simulink model "SimulationMain"  (R2023b)
settings: Solver=FixedStepAuto  StartTime=0.0  StopTime=Inf  RelTol=1e-3
undefined symbols (not defined in the file): ADC_VMax, ADC_VMin, CurrentSensor_Bias, CurrentSensor_Gain, DC_V, DiscIntNeverNeededParam, DoorStairOutTime1, DoorStairOutTime2, FloorHeight, FloorStairOut, FloorTimeStairOut, IO397, Omega2RPM, Pulley, StairOutTime1, StairOutTime2
libraries: fl_lib x10, ee_lib x10, nesl_utility x8, mcbplantlib x1, speedgoatlib_fpga x1, speedgoatlib_fpga_analog_io x1, speedgoatlib_fpga_quadrature x1, speedgoatlib_fpga_pwm x1
settings Model: DataDictionary=Data_GeneralDefinition.sldd  Creator=rodri  LastModifiedBy=rodri
settings SolverCC: ConcurrentTasks=on  PositivePriorityOrder=on
settings OptimizationCC: BlockReduction=off  OptimizeBlockIOStorage=off
settings DebuggingCC: TasksWithSamePriorityMsg=none
settings HardwareCC: ProdBitPerLong=64  ProdLongLongMode=on  ProdHWDeviceType=Intel->x86-64 (Linux 64)
settings ModelReferenceCC: ModelReferenceNumInstancesAllowed=Single
settings RTWCC: Description=Simulink Real-Time  SystemTargetFile=slrealtime.tlc  TemplateMakefile=slrealtime_default_tmf  Toolchain=Simulink Real-Time Toolchain  BuildConfiguration=Faster Runs  CodeExecutionProfiling=on  TargetLang=C++
settings ExplorerConfigSet: SimMechanicsOpenEditorOnUpdate=off

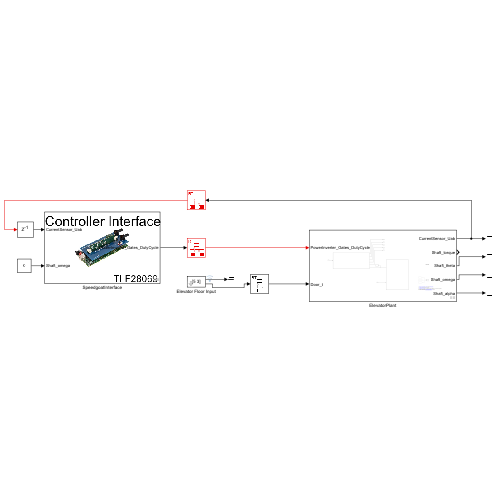
[thumbnail: Simulink's stored preview of the top-level diagram]
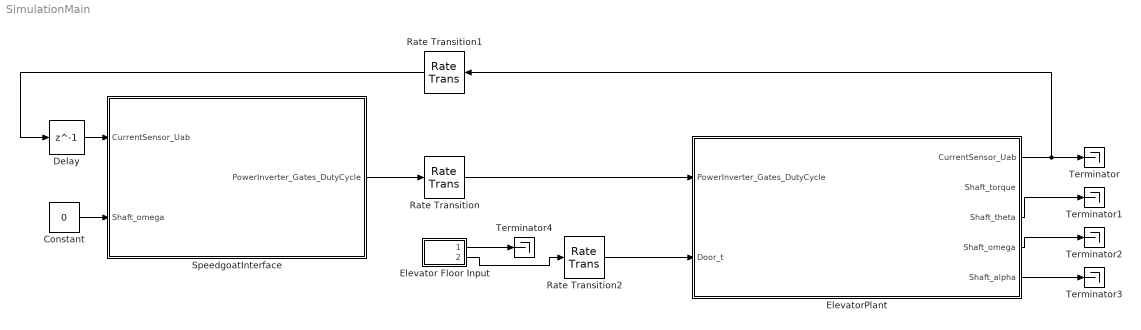
== system SimulationMain ==
  Constant : Constant  Value=0  SampleTime=-1
  Delay : Delay  DelayLength=1
  Elevator Floor Input : Subsystem  mask(Elevator Floors Input){FloorNums=[5 3]}
      mask prompts: FloorNums "Enter Floor Numbers"
      mask help:
      | Provide the floor numbers (1 to 7) for the elevator. This should be a (1 x n) vector. (n<=3)
      |
      | For example, an input of [4 2] means the elevator will go to the 4th Floor first and then the 2nd Floor.
      mask init:
      | if ~isrow(str2num(get_param(gcb,'FloorNums')))
      |     error('Input should be a row vector');
      | end
      | 
      | if length(str2num(get_param(gcb,'FloorNums')))>3
      |     error('Length of input row vector should not be greater then 3');
      | end
      | 
      | if any(str2num(get_param(gcb,'FloorNums'))>7)
      |     error('Elevator can not go above 7 floors for this system');
      | end
      | 
      | if any(str2num(get_param(gcb,'FloorNums'))<=0)
      |     error('Elevator floor input should be greater then 0');
      | end
      mask Display: disp(get_param(gcb,'FloorNums'));
  ElevatorPlant : Subsystem
  Rate Transition : RateTransition
  Rate Transition1 : RateTransition
  Rate Transition2 : RateTransition
  SpeedgoatInterface : Subsystem
  Terminator{,1..4} (5 alike) : Terminator
  wires:
  SpeedgoatInterface/1(PowerInverter_Gates_DutyCycle) -> Rate Transition/1
  Constant/1 -> SpeedgoatInterface/2(Shaft_omega)
  ElevatorPlant/1(CurrentSensor_Uab) -> Rate Transition1/1, Terminator/1
  ElevatorPlant/3(Shaft_theta) -> Terminator1/1
  ElevatorPlant/4(Shaft_omega) -> Terminator2/1
  ElevatorPlant/5(Shaft_alpha) -> Terminator3/1
  Delay/1 -> SpeedgoatInterface/1(CurrentSensor_Uab)
  Rate Transition/1 -> ElevatorPlant/1(PowerInverter_Gates_DutyCycle)
  Rate Transition1/1 -> Delay/1
  Elevator Floor Input/2(DoorOperationTimes) -> Rate Transition2/1
  Elevator Floor Input/1(MotorMotion) -> Terminator4/1
  Rate Transition2/1 -> ElevatorPlant/2(Door_t)

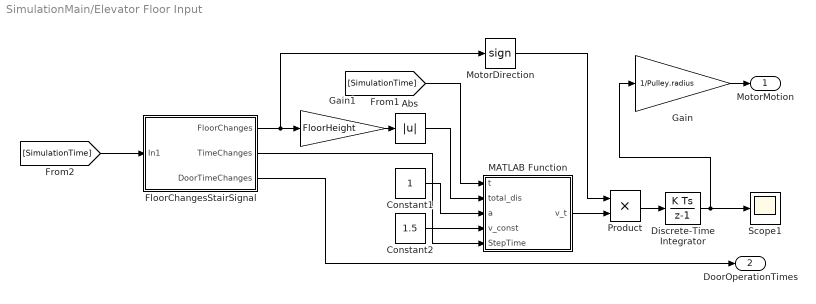
== system SimulationMain/Elevator Floor Input ==
  Abs : Abs  SaturateOnIntegerOverflow=off
  Constant1 : Constant  SampleTime=-1
  Constant2 : Constant  Value=1.5  SampleTime=-1
  Discrete-Time Integrator : DiscreteIntegrator  SampleTime=-1  ICPrevOutput=DiscIntNeverNeededParam  ICPrevScaledInput=DiscIntNeverNeededParam
  FloorChangesStairSignal : Subsystem  mask{FloorNums=FloorNums}
      mask prompts: FloorNums "Enter Floor Nums for Elevator"
      mask init:
      | [FloorStairOut,FloorTimeStairOut,StairOutTime1,StairOutTime2,DoorStairOutTime1,DoorStairOutTime2]...
      |  = getLookUpTableData(FloorNums);
  Gain : Gain  Gain=1/Pulley.radius
  Gain1 : Gain  Gain=FloorHeight
  MATLAB Function : MATLAB Function  TreatAsAtomicUnit=on
  MotorDirection : Signum
  Product : Product
  Scope1 : Scope
  MotorMotion : Outport  VectorParamsAs1DForOutWhenUnconnected=off
  DoorOperationTimes : Outport  Port=2  VectorParamsAs1DForOutWhenUnconnected=off
  wires:
  FloorChangesStairSignal/3(DoorTimeChanges) -> DoorOperationTimes/1
  Abs/1 -> MATLAB Function/2(total_dis)
  FloorChangesStairSignal/1(FloorChanges) -> MotorDirection/1, Gain1/1
  FloorChangesStairSignal/2(TimeChanges) -> MATLAB Function/5(StepTime)
  MATLAB Function/1(v_t) -> Product/2
  Product/1 -> Discrete-Time Integrator/1
  MotorDirection/1 -> Product/1
  Gain/1 -> MotorMotion/1
  Gain1/1 -> Abs/1
  [SimulationTime] -> MATLAB Function/1(t)
  Constant1/1 -> MATLAB Function/3(a)
  Constant2/1 -> MATLAB Function/4(v_const)
  Discrete-Time Integrator/1 -> Scope1/1, Gain/1
  [SimulationTime] -> FloorChangesStairSignal/1(In1)

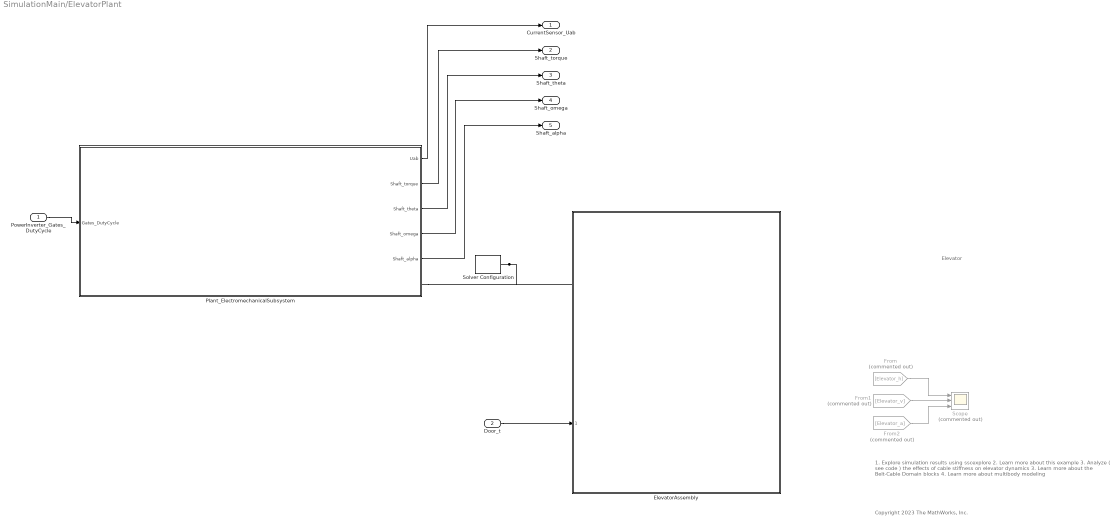
== system SimulationMain/ElevatorPlant ==
  note: 1. Explore simulation results using sscexplore
      | 2. Learn more about this example
      | 3. Analyze ( see code ) the effects of cable stiffness on elevator dynamics
      | 3. Learn more about the Belt-Cable Domain blocks
      | 4. Learn more about multibody modeling
  note: Elevator
  note: Copyright 2023 The MathWorks, Inc.
  PowerInverter_Gates_DutyCycle : Inport
  Door_t : Inport  Port=2
  ElevatorAssembly : Subsystem  ReferencedSubsystem=ElevatorAssembly
      settings: PortSchema="{\"entries\":[{\"content\":{\"sides\":[{\"content\":{\"connectorIds\":[\"LConn1\",\"In1\"]},\"type\":\"ConnectorPlacement.EquallySpacedRectSide\",\"uuid\":\"d6cdcc45-76f5-4e8f-aa72-f7931a260e9d\"},{\"content\":{\"side\":\"RIGHT\"},\"type\":\"ConnectorPlacement.EquallySpacedRectSide\",\"uuid\":\"7886d4e3-3d61-4781-ae6a-17f03b8e636c\"},{\"content\":{\"side\":\"TOP\"},\"type\":\"ConnectorPlacement.EquallySpacedRectSide\",\"uuid\":\"a03356aa-ba1a-42a9-a233-3323839a0ec6\"}]},\"type\":\"ConnectorPlacement.EquallySpacedConnector\",\"uuid\":\"80b5650e-2a4d-4b3a-8116-45d32f4901f0\"}],\"packageUris\":[\"http://schema.mathworks.com/mf0/Connector/R2020b\"],\"version\":\"1.0\"}"
  From : From  Commented=on  GotoTag=Elevator_h  TagVisibility=global
  From1 : From  Commented=on  GotoTag=Elevator_v  TagVisibility=global
  From2 : From  Commented=on  GotoTag=Elevator_a  TagVisibility=global
  Plant_ElectromechanicalSubsystem : Subsystem
  Scope : Scope  Commented=on  NumInputPorts=3
  Solver Configuration : nesl_utility/Solver Configuration  PhysicalDomain=network_engine_domain  SubClassName=solver  LeftPortType=input  RightPortType=generic  Tones=[]  Harmonics=[]  SimulateNoise=off  Profile=off  UseLocalSampling=off  EnableSwitchedLinearOptims=on  FrequencyDomain=off  UseCCode=off  RelTol=0.001  AbsTol=0.001  MinStep=1e-09  ToWorkspace=off  RevertToSquareIcSolve=off  NumHomotopyIterations=100  PhasorMode=off  PhasorModeNumHarmonics=1  ConsistencySolver=NEWTON_XTOL_AFTER_FTOL  IndexReductionMethod=DerivativeReplacement  DoDC=off  ResidualTolerance=1e-09  ConsistencyTolSource=GLOBAL  ConsistencyAbsTol=0.001  ConsistencyRelTol=0.001  ConsistencyTolFactor=0.001  UseLocalSolver=on  LocalSolverChoice=NE_BACKWARD_EULER_ADVANCER  ResolveIndetEquations=on  FunctionEvalNumThread=1  LocalSolverSampleTime=0.002  DoFixedCost=on  MaxNonlinIter=3  MaxModeIter=2  ComputeImpulses=off  ImpulseIterations=2  LinearAlgebra=auto  LinearAlgebraNumThread=0  EquationFormulation=NE_TIME_EF  DelaysMemoryBudget=1024  AutomaticFiltering=on  FilteringTimeConstant=0.001  PartitionStorageMethod=AS_NEEDED  PartitionMemoryBudget=1024  PartitionMethod=ROBUST  MultibodyUseLocalSolver=off  MultibodyLocalSolverChoice=ODE1  MultibodyLocalSolverSampleTime=0.001
  CurrentSensor_Uab : Outport
  Shaft_torque : Outport  Port=2
  Shaft_theta : Outport  Port=3
  Shaft_omega : Outport  Port=4
  Shaft_alpha : Outport  Port=5
  wires:
  Plant_ElectromechanicalSubsystem/5(Shaft_alpha) -> Shaft_alpha/1
  Plant_ElectromechanicalSubsystem/4(Shaft_omega) -> Shaft_omega/1
  Plant_ElectromechanicalSubsystem/3(Shaft_theta) -> Shaft_theta/1
  Plant_ElectromechanicalSubsystem/2(Shaft_torque) -> Shaft_torque/1
  Plant_ElectromechanicalSubsystem/1(Uab) -> CurrentSensor_Uab/1
  PowerInverter_Gates_DutyCycle/1 -> Plant_ElectromechanicalSubsystem/1(Gates_DutyCycle)
  From/1 -> Scope/1
  From1/1 -> Scope/2
  From2/1 -> Scope/3
  Door_t/1 -> ElevatorAssembly/1
  connections:
  Solver Configuration/RConn1 -- ElevatorAssembly/LConn1 -- Plant_ElectromechanicalSubsystem/RConn1

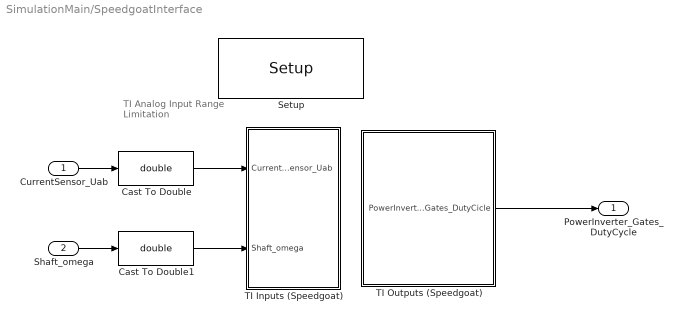
== system SimulationMain/SpeedgoatInterface ==
  note: TI Analog Input Range Limitation
  CurrentSensor_Uab : Inport  OutDataTypeStr=double  PortDimensions=2
  Shaft_omega : Inport  Port=2  OutDataTypeStr=double  PortDimensions=1
  Cast To Double : DataTypeConversion  OutMin=ADC_VMin  OutMax=ADC_VMax  OutDataTypeStr=double  SaturateOnIntegerOverflow=off  RndMeth=Floor
  Cast To Double1 : DataTypeConversion  OutDataTypeStr=double  SaturateOnIntegerOverflow=off  RndMeth=Floor
  Setup : speedgoatlib_fpga/Setup/Setup  board=IO397-50k  id=1  device_id=1  frontIO=None  rearIO=None  bitstreamFile=speedgoat_IO397_HIL.mat  rev=7.100000  timestamp_string=04/06/24 08:23:17  fpgaFreq=75 MHz  fpgaTick=13.33 ns  ProgSpiFlash=off  ProgBPIFlash=off  pciSlot=-1  useFpgaDmaController=off  PullRPort0=pull-up 3.3V  VioPort0=3.3V  PullRPort1=pull-up 3.3V  VioPort1=3.3V  PullRPort2=pull-up 3.3V  VioPort2=3.3V  PullRPort3=pull-up 3.3V  VioPort3=3.3V  PullRPort4=pull-up 3.3V  VioPort4=3.3V  PullRPort5=pull-up 3.3V  VioPort5=3.3V  PullRPort6=pull-up 3.3V  VioPort6=3.3V  diffLineTermination_rear1=on  diffLineTermination_rear2=on  diffLineTermination_rear3=on  diffLineTermination_rear4=on  diffLineTermination_rear5=on  diffLineTermination_rear6=on  diffLineTermination_rear7=on  diffLineTermination_rear8=on  PullRPort15=pull-up 3.3V  PullRPort31=pull-up 3.3V  PullRPort47=pull-up 3.3V  PullRPort63=pull-up 3.3V  diffLineTermination_1=on  diffLineTermination_2=on  diffLineTermination_3=on  diffLineTermination_4=on  diffLineTermination_5=on  diffLineTermination_6=on  diffLineTermination_7=on  diffLineTermination_8=on  diffLineTermination_9=on  diffLineTermination_10=on  diffLineTermination_11=on  diffLineTermination_12=on  diffLineTermination_13=on  diffLineTermination_14=on  diffLineTermination_15=on  diffLineTermination_16=on  diffLineTermination_17=on  diffLineTermination_18=on  diffLineTermination_19=on  diffLineTermination_20=on  diffLineTermination_21=on  diffLineTermination_22=on  diffLineTermination_23=on  diffLineTermination_24=on  diffLineTermination_25=on  diffLineTermination_26=on  diffLineTermination_27=on  diffLineTermination_28=on  diffLineTermination_29=on  diffLineTermination_30=on  diffLineTermination_31=on  diffLineTermination_32=on  Vo_36x_1=3.3V  Vi_Pull_36x_1=Floating  Vo_36x_2=3.3V  Vi_Pull_36x_2=Floating  Vo_36x_3=3.3V  Vi_Pull_36x_3=Floating  Vo_36x_4=3.3V  Vi_Pull_36x_4=Floating  Vo_36x_5=3.3V  Vi_Pull_36x_5=Floating  Vo_36x_6=3.3V  Vi_Pull_36x_6=Floating  Vo_36x_7=3.3V  Vi_Pull_36x_7=Floating  Vo_36x_8=3.3V  Vi_Pull_36x_8=Floating  Vo_36x_9_16=3.3V  Vi_Pull_36x_9_16=Floating  Vo_36x_17_24=3.3V  Vi_Pull_36x_17_24=Floating  Vo_36x_25_32=3.3V  Vi_Pull_36x_25_32=Floating  Vo_36x_33_40=3.3V  Vi_Pull_36x_33_40=Floating  Vo_36x_41_48=3.3V  Vi_Pull_36x_41_48=Floating  Vo_36x_49_56=3.3V  Vi_Pull_36x_49_56=Floating  Vo_36x_57_64=3.3V  Vi_Pull_36x_57_64=Floating
      settings: SourceProductName=Simulink Real-Time: Speedgoat I/O Blockset
  TI Inputs (Speedgoat) : Subsystem
  TI Outputs (Speedgoat) : Subsystem
  PowerInverter_Gates_DutyCycle : Outport  OutDataTypeStr=double  PortDimensions=6
  wires:
  Cast To Double1/1 -> TI Inputs (Speedgoat)/2(Shaft_omega)
  CurrentSensor_Uab/1 -> Cast To Double/1
  Shaft_omega/1 -> Cast To Double1/1
  Cast To Double/1 -> TI Inputs (Speedgoat)/1(CurrentSensor_Uab)
  TI Outputs (Speedgoat)/1(PowerInverter_Gates_DutyCicle) -> PowerInverter_Gates_DutyCycle/1

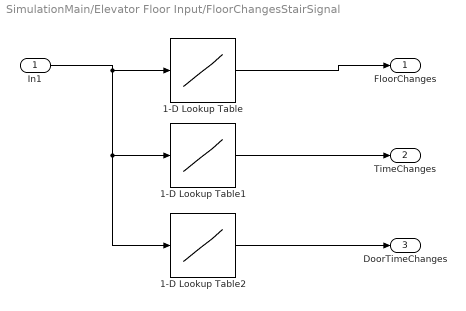
== system SimulationMain/Elevator Floor Input/FloorChangesStairSignal ==
  In1 : Inport
  1-D Lookup Table : Lookup_n-D  NumberOfTableDimensions=1  BreakpointsForDimension1=FloorTimeStairOut  BreakpointsForDimension1FirstPoint=2  Table=FloorStairOut  ExtrapMethod=Clip  UseLastTableValue=on  InternalRulePriority=Speed  RndMeth=Nearest
  1-D Lookup Table1 : Lookup_n-D  NumberOfTableDimensions=1  BreakpointsForDimension1=StairOutTime2  BreakpointsForDimension1FirstPoint=2  Table=StairOutTime1  ExtrapMethod=Clip  UseLastTableValue=on  InternalRulePriority=Speed  RndMeth=Nearest
  1-D Lookup Table2 : Lookup_n-D  NumberOfTableDimensions=1  BreakpointsForDimension1=DoorStairOutTime2  BreakpointsForDimension1FirstPoint=2  Table=DoorStairOutTime1  ExtrapMethod=Clip  UseLastTableValue=on  InternalRulePriority=Speed  RndMeth=Nearest
  FloorChanges : Outport  VectorParamsAs1DForOutWhenUnconnected=off
  TimeChanges : Outport  Port=2  VectorParamsAs1DForOutWhenUnconnected=off
  DoorTimeChanges : Outport  Port=3  VectorParamsAs1DForOutWhenUnconnected=off
  wires:
  In1/1 -> 1-D Lookup Table2/1, 1-D Lookup Table1/1, 1-D Lookup Table/1
  1-D Lookup Table/1 -> FloorChanges/1
  1-D Lookup Table1/1 -> TimeChanges/1
  1-D Lookup Table2/1 -> DoorTimeChanges/1

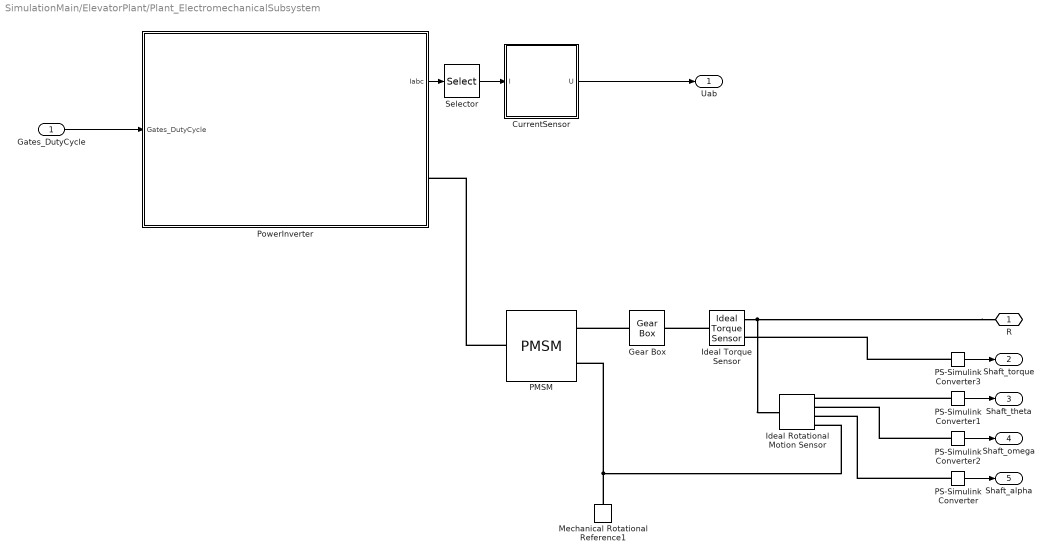
== system SimulationMain/ElevatorPlant/Plant_ElectromechanicalSubsystem ==
  Gates_DutyCycle : Inport
  CurrentSensor : Subsystem
  Gear Box : fl_lib/Mechanical/Mechanisms/Gear Box  ratio=10  t_in_specify=off  t_in_priority=None  t_in=0 N*m  t_in_nominal_specify=off  t_in_nominal_unit=N*m  t_in_nominal_value=1  t_out_specify=off  t_out_priority=None  t_out=0 N*m  t_out_nominal_specify=off  t_out_nominal_unit=N*m  t_out_nominal_value=1
  Ideal Rotational Motion Sensor : fl_lib/Mechanical/Mechanical Sensors/Ideal Rotational Motion Sensor  reference=foundation.enum.MeasurementReference.difference  acceleration_port=true  velocity_port=true  position_port=true  wrap_angle=false  offset=0 rad
      settings: InternalSimscapePortConfiguration="{\"Bottom\":[],\"Left\":[{\"id\":\"R\",\"label\":\"R\",\"type\":\"foundation.mechanical.rotational.rotational\"}],\"Right\":[{\"id\":\"C\",\"label\":\"C\",\"type\":\"foundation.mechanical.rotational.rotational\"},{\"id\":\"alpha\",\"label\":\"α\",\"type\":\"output\"},{\"id\":\"W\",\"label\":\"W\",\"type\":\"output\"},{\"id\":\"A\",\"label\":\"A\",\"type\":\"output\"}],\"Top\":[]}"
  Ideal Torque Sensor : fl_lib/Mechanical/Mechanical Sensors/Ideal Torque Sensor
  Mechanical Rotational Reference1 : fl_lib/Mechanical/Rotational Elements/Mechanical Rotational Reference
  PMSM : ee_lib/Electromechanical/Permanent Magnet/PMSM  Tag={'toolbox/physmod/elec/library/m/ee_lib_parts';'Electromechanical/Permanent_Magnet/PMSM/Siemens/x1FT7108_5AC7.xml'}  port_option=ee.enum.threePhasePort.composite  winding_type=ee.enum.statorconnection.wye  machine_param=ee.enum.pmsm.parameterization.constant  nPolePairs=5  pmflux_param=ee.enum.pmflux.fluxlinkage  pm_flux_linkage=0.270554790028086 Wb  torque_constant=1.35277395014043 N*m/A  back_emf_constant=1.35277395014043 V/(rad/s)  stator_param=ee.enum.statorparam.LdLqL0  Ld=0.0031 H  Lq=0.0031 H  idVec=[-200 0 200] % Parameter not set A  iqVec=[-200 0 200] % Parameter not set A  LdMatrix=[0.0002 0.0002 0.0002;0.0002 0.0002 0.0002;0.0002 0.0002 0.0002] % Parameter not set H  LqMatrix=[0.0002 0.0002 0.0002;0.0002 0.0002 0.0002;0.0002 0.0002 0.0002] % Parameter not set H  PmMatrix=[0.1 0.1 0.1;0.1 0.1 0.1;0.1 0.1 0.1] Wb  ktMatrix=[0.18 0.18 0.18;0.18 0.18 0.18;0.18 0.18 0.18] N*m/A  keMatrix=[0.18 0.18 0.18;0.18 0.18 0.18;0.18 0.18 0.18] % Parameter not set V/(rad/s)  L0=[] % Parameter not set H  Ls=0.0002 H  Lm=-2e-05 H  Ms=2e-05 H  Rs=0.111 Ohm  zero_sequence=ee.enum.park.zerosequence.exclude  axes_param=ee.enum.rotorangle.daxis  loss_param=ee.enum.ironloss.none  losses_oc=[0 0 0] % Parameter not set W  losses_sc=[0 0 0] % Parameter not set W  f_losses=60 % Parameter not set Hz  Isc_losses=95 % Parameter not set A  J=0.0248 kg*m^2  lam=0 % Parameter not set N*m/(rad/s)  i_d_specify=off  i_d_priority=None  i_d=0 A  i_d_nominal_specify=off  i_d_nominal_unit=A  i_d_nominal_value=1  i_q_specify=off  i_q_priority=None  i_q=0 A  i_q_nominal_specify=off  i_q_nominal_unit=A  i_q_nominal_value=1  torque_specify=off  torque_priority=None  torque=0 N*m  torque_nominal_specify=off  torque_nominal_unit=N*m  torque_nominal_value=1  angular_velocity_specify=off  angular_velocity_priority=High  angular_velocity=0 rpm  angular_velocity_nominal_specify=off  angular_velocity_nominal_unit=rpm  angular_velocity_nominal_value=1  angular_position_specify=off  angular_position_priority=High  angular_position=0 deg  angular_position_nominal_specify=off  angular_position_nominal_unit=deg  angular_position_nominal_value=1  alpha=3.93e-3 1/K  alpha_flux=-0.001 1/K  Tmeas=298.15 K  stator_thermal_mass=100 J/K  rotor_thermal_mass=200 J/K  Rm_percent_rotor=90  Rd_percent_rotor=30  temperatureA_specify=off  temperatureA_priority=High  temperatureA=25 degC  temperatureA_nominal_specify=off  temperatureA_nominal_unit=degC  temperatureA_nominal_value=1  temperatureB_specify=off  temperatureB_priority=High  temperatureB=25 degC  temperatureB_nominal_specify=off  temperatureB_nominal_unit=degC  temperatureB_nominal_value=1  temperatureC_specify=off  temperatureC_priority=High  temperatureC=25 degC  temperatureC_nominal_specify=off  temperatureC_nominal_unit=degC  temperatureC_nominal_value=1  temperatureR_specify=off  temperatureR_priority=High  temperatureR=25 degC  temperatureR_nominal_specify=off  temperatureR_nominal_unit=degC  temperatureR_nominal_value=1
      settings: AttributesFormatString=Siemens:1FT7108-5AC7  InternalSimscapePortConfiguration="{\"Bottom\":[],\"Left\":[{\"id\":\"N\",\"label\":\"~\",\"type\":\"foundation.electrical.three_phase\"}],\"Right\":[{\"id\":\"R\",\"label\":\"R\",\"type\":\"foundation.mechanical.rotational.rotational\"},{\"id\":\"C\",\"label\":\"C\",\"type\":\"foundation.mechanical.rotational.rotational\"}],\"Top\":[]}"
  PS-Simulink Converter{,1..3} (4 alike) : nesl_utility/PS-Simulink Converter  PhysicalDomain=network_engine_domain  SubClassName=ps_output  LeftPortType=input  RightPortType=output  PseudoPeriodic=off  Frequencies=[]  VectorFormat=inherit  Unit=inherit  AffineConversion=off
  PowerInverter : Subsystem
  Selector : Selector  InputPortWidth=3  IndexOptions=Index vector (dialog)  Indices=[1 2]  OutputSizes=1
  R : PMIOPort  Side=Right
  Uab : Outport
  Shaft_torque : Outport  Port=2
  Shaft_theta : Outport  Port=3
  Shaft_omega : Outport  Port=4
  Shaft_alpha : Outport  Port=5
  wires:
  PS-Simulink Converter3/1 -> Shaft_torque/1
  PS-Simulink Converter/1 -> Shaft_alpha/1
  PS-Simulink Converter2/1 -> Shaft_omega/1
  PS-Simulink Converter1/1 -> Shaft_theta/1
  Selector/1 -> CurrentSensor/1(I)
  PowerInverter/1(Iabc) -> Selector/1
  Gates_DutyCycle/1 -> PowerInverter/1(Gates_DutyCycle)
  CurrentSensor/1(U) -> Uab/1
  connections:
  Ideal Torque Sensor/LConn1 -- Gear Box/RConn1
  PS-Simulink Converter3/LConn1 -- Ideal Torque Sensor/RConn2
  Gear Box/LConn1 -- PMSM/RConn1
  PS-Simulink Converter1/LConn1 -- Ideal Rotational Motion Sensor/RConn4
  PS-Simulink Converter2/LConn1 -- Ideal Rotational Motion Sensor/RConn3
  PS-Simulink Converter/LConn1 -- Ideal Rotational Motion Sensor/RConn2
  PMSM/LConn1 -- PowerInverter/RConn1
  PMSM/RConn2 -- Ideal Rotational Motion Sensor/RConn1 -- Mechanical Rotational Reference1/LConn1
  R/RConn1 -- Ideal Rotational Motion Sensor/LConn1 -- Ideal Torque Sensor/RConn1

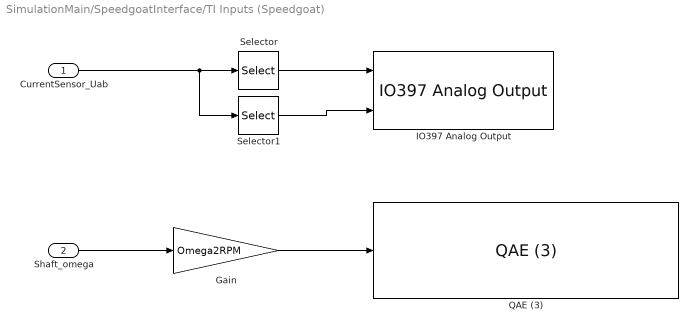
== system SimulationMain/SpeedgoatInterface/TI Inputs (Speedgoat) ==
  CurrentSensor_Uab : Inport
  Shaft_omega : Inport  Port=2
  Gain : Gain  Gain=Omega2RPM
  IO397 Analog Output : speedgoatlib_fpga_analog_io/IO397 Analog Output  id=1  chan=[1 2]  initVal=0  resetVal=0  ts=0.002  span=+5 V
      settings: SourceProductName=Simulink Real-Time: Speedgoat I/O Blockset
  QAE (3) : speedgoatlib_fpga_quadrature/QAE (3)  id=1  chan=[1]  sampleTime=0.002  enableDma=on  numOfSlots=[16]  sigAswitchOn=[180]  sigBswitchOff=[90]  sigBswitchOn=[270]  initPos=0  sigAdismissEn=off  sigAdismissSingle=on  sigAdismissHigh=on  sigBdismissEn=off  sigBdismissSingle=on  sigBdismissHigh=on  showOutputPosition=off  showOutputSlotAngle=off
      settings: SourceProductName=Simulink Real-Time: Speedgoat I/O Blockset
  Selector : Selector  InputPortWidth=2  IndexOptions=Index vector (dialog)  Indices=1  OutputSizes=1
  Selector1 : Selector  InputPortWidth=2  IndexOptions=Index vector (dialog)  Indices=2  OutputSizes=1
  wires:
  CurrentSensor_Uab/1 -> Selector1/1, Selector/1
  Shaft_omega/1 -> Gain/1
  Selector/1 -> IO397 Analog Output/1
  Selector1/1 -> IO397 Analog Output/2
  Gain/1 -> QAE (3)/1

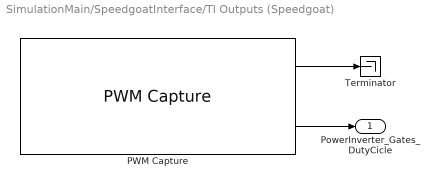
== system SimulationMain/SpeedgoatInterface/TI Outputs (Speedgoat) ==
  PWM Capture : speedgoatlib_fpga_pwm/PWM Capture  id=1  chan=[2 6 4 1 5 3 ]  ts=0.002  enableDma=on  captureMode=High transitions triggered  bit_width_cap=24  captureTimeout_si=0  captureTimeout_eff=0  captureTimeout=0  debounce_si=10e-6  debounce_eff=10e-6  debounce=750  showHighDuration=off  showLowDuration=off  showPeriod=on  showDC16=on  showDC8=off  showTOn=off  showTOff=off  showValidData=off
      settings: SourceProductName=Simulink Real-Time: Speedgoat I/O Blockset
  Terminator : Terminator
  PowerInverter_Gates_DutyCicle : Outport
  wires:
  PWM Capture/2 -> PowerInverter_Gates_DutyCicle/1
  PWM Capture/1 -> Terminator/1

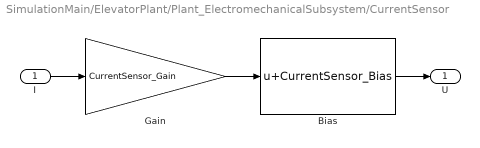
== system SimulationMain/ElevatorPlant/Plant_ElectromechanicalSubsystem/CurrentSensor ==
  I : Inport
  Bias : Bias  Bias=CurrentSensor_Bias  SaturateOnIntegerOverflow=off
  Gain : Gain  Gain=CurrentSensor_Gain
  U : Outport
  wires:
  I/1 -> Gain/1
  Gain/1 -> Bias/1
  Bias/1 -> U/1

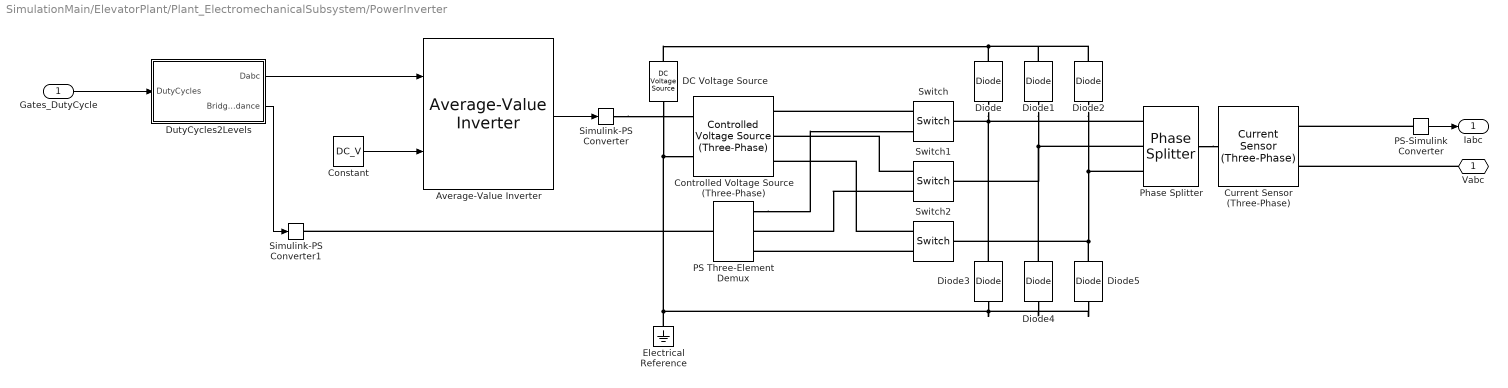
== system SimulationMain/ElevatorPlant/Plant_ElectromechanicalSubsystem/PowerInverter ==
  Gates_DutyCycle : Inport
  Average-Value Inverter : mcbplantlib/Average-Value Inverter
      settings: LibrarySourceBlock=mcblib/Electrical Systems/Inverters/Average-Value Inverter
  Constant : Constant  Value=DC_V
  Controlled Voltage Source (Three-Phase) : ee_lib/Sources/Controlled Voltage Source (Three-Phase)  input_option=ee.enum.inputType.instantaneous  FRated=60 Hz
      settings: InternalSimscapePortConfiguration="{\"Bottom\":[],\"Left\":[{\"id\":\"S\",\"label\":\"S\",\"type\":\"input\"},{\"id\":\"n\",\"label\":\"n\",\"type\":\"foundation.electrical.electrical\"}],\"Right\":[{\"id\":\"a\",\"label\":\"a\",\"type\":\"foundation.electrical.electrical\"},{\"id\":\"b\",\"label\":\"b\",\"type\":\"foundation.electrical.electrical\"},{\"id\":\"c\",\"label\":\"c\",\"type\":\"foundation.electrical.electrical\"}],\"Top\":[]}"
  Current Sensor (Three-Phase) : ee_lib/Sensors & Transducers/Current Sensor (Three-Phase)
  DC Voltage Source : fl_lib/Electrical/Electrical Sources/DC Voltage Source  v0=DC_V V
  Diode{,1..5} (6 alike) : ee_lib/Semiconductors & Converters/Diode  ModelType=ee.enum.diode.modelType.pwl  TableType=ee.enum.diode.tableType.IfMat  IfMat=[.07, .12, .19, 1.75, 4.24, 7.32, 11.2; .16, .3, .72, 2.14, 5.02, 8.35, 13.12] A  VfMat=[.9, 1.15, 1.25, 1.5, 1.75, 2.17, 2.6, 2.85; .58, .68, .75, 1.1, 1.38, 1.77, 2.27, 2.7] V  TjVec=[25, 125] degC  VfVec=[.5, .7, .9, 1.3, 1.7, 2.1, 2.5] V  IfVec=[.1, .2, .5, 1, 2, 4, 7, 10] A  Vf=0.6 V  Ron=0.3 Ohm  Goff=1e-8 S  prmExp=ee.enum.diode.expParam.useTwo  I12=[.0137, .545] A  V12=[.6, .7] V  RS=0 Ohm  Tmeas=25 degC  IS=1e-12 A  ec=1  I1=0.0137 A  V1=0.6 V  N_series=1  N_parallel=1  ZenerEnable=false  Rz=0.3 Ohm  BV=inf V  C_param=ee.enum.diode.capParam.fixed  CJ=0 pF  CJ0=5 pF  Vvec=[.1, 10, 100] V  Cvec=[3.5, 1, .4] pF  VJ=1 V  Mgrad=0.5  FC=0.5  Q_param=ee.enum.diode.recoveryParam.off  iRM=-7.15 A  iF=4 A  didt=-750 A/us  trr_factor=3  trr=115 ns  Qrr=150 nA*s  Vr=-600 V  Ls=150 nH  Erec=0.03 J  TT=50 ns  tau=100 ns  T_param=ee.enum.diode.temperatureParam.off  Tdevice=25 degC  I1_T2=0.245 A  V1_T2=0.5 V  IS_T2=1.25e-7 A  Tmeas2=125 degC  XTI_param=ee.enum.diode.xtiParam.pn  XTI=3  EG_param=ee.enum.diode.egapParam.material_si  EG=1.11 eV  dBVdT=0 V/K  enable_faults=simscape.enum.onoff.off  fault_action=simscape.enum.assert.action.none  fault_types=ee.enum.diode.faults.open  tau_fault=1e-3 s  IfMat_faulted=[.07, .12, .19, 1.75, 4.24, 7.32, 11.2; .16, .3, .72, 2.14, 4.02, 6.35, 9.12] A  VfMat_faulted=[.9, 1.15, 1.25, 1.5, 1.75, 2.17, 2.6, 2.85; .58, .68, .75, 1.1, 1.38, 1.77, 2.27, 2.7] V  VfVec_faulted=[.5, .7, .9, 1.3, 1.7, 2.1, 2.5] V  IfVec_faulted=[.1, .2, .5, 1, 2, 4, 7, 10] A  Ropen_faulted=1000 Ohm  Gshort_faulted=1000 1/Ohm  Vf_faulted=0.6 V  Ron_faulted=0.3 Ohm  Goff_faulted=1e-8 S  I12_faulted=[.0137, .545] A  V12_faulted=[.6, .7] V  IS_faulted=1e-12 A  ec_faulted=1  I1_faulted=0.0137 A  V1_faulted=0.6 V  RS_faulted=0 Ohm  Rz_faulted=0.3 Ohm  BV_faulted=inf V  Cscale_faulted=100  fault_trigger=ee.enum.faults.faultTrigger.temporal  t_fault=inf s  max_permissible_voltage=inf V  n_fail_on_voltage=1  max_permissible_current=inf A  t_fail_on_current=1 s  max_permissible_dVdt=inf V/s  enable_fault_input=simscape.enum.onoff.off  i_specify=off  i_priority=None  i=0 A  i_nominal_specify=off  i_nominal_unit=A  i_nominal_value=1  v_specify=off  v_priority=None  v=0 V  v_nominal_specify=off  v_nominal_unit=V  v_nominal_value=1  v_capacitor_specify=off  v_capacitor_priority=None  v_capacitor=0 V  v_capacitor_nominal_specify=off  v_capacitor_nominal_unit=V  v_capacitor_nominal_value=1  faulted_specify=off  faulted_priority=None  faulted=0  faulted_nominal_specify=off  faulted_nominal_unit=1  faulted_nominal_value=1  i_diode_specify=off  i_diode_priority=None  i_diode=0 A  i_diode_nominal_specify=off  i_diode_nominal_unit=A  i_diode_nominal_value=1  v_diode_specify=off  v_diode_priority=None  v_diode=0 V  v_diode_nominal_specify=off  v_diode_nominal_unit=V  v_diode_nominal_value=1  i_capacitor_specify=off  i_capacitor_priority=None  i_capacitor=0 A  i_capacitor_nominal_specify=off  i_capacitor_nominal_unit=A  i_capacitor_nominal_value=1  power_dissipated_specify=off  power_dissipated_priority=None  power_dissipated=0 W  power_dissipated_nominal_specify=off  power_dissipated_nominal_unit=W  power_dissipated_nominal_value=1  fidelity_level=ee.enum.diode.fidelity.includeChargeDyn  rec_loss_model=ee.enum.diode.reverseRecoveryModel.fixed  ErecVal=0 J  scaleWithIandV=true  ErecMat=zeros(2, 3) J  TjrecVec=[298.15, 398.15] K  IfrecVec=[.1, 1, 10] A  IrecVal=10 A  VrecVal=10 V  tFilter=1 / 1000 / 100 s  max_permissible_temperature=inf K  t_fail_on_temperature=1 s  thermal_network_parameterization=ee.enum.thermalNetworkTopology.junctionCase  Rth=[0, 10] K/W  Rth_Cauer=[1, 3, 10] K/W  Rth_Foster=[4, 6] K/W  thermal_mass_parameterization=ee.enum.thermalNetwork.timeconstant  thermal_mass=[0, 1] J/K  thermal_mass_Cauer=[.1, .3, 1] J/K  thermal_mass_Foster=[1.5, 3] J/K  thermal_time_constant=[0, 10] s  thermal_time_constant_Cauer=[1, 3, 10] s  thermal_time_constant_Foster=[6, 18] s  thermal_mass_initial_temperatures=[25, 25] degC  thermal_mass_initial_temperatures_Cauer=[25, 25, 25] degC  junction_thermal_mass=0.01 J/K  Tvec_initial_Foster=[25, 25, 25, 25] degC  no_thermal_network=0  junction_temperature_specify=off  junction_temperature_priority=None  junction_temperature=25 degC  junction_temperature_nominal_specify=off  junction_temperature_nominal_unit=degC  junction_temperature_nominal_value=1
  DutyCycles2Levels : Subsystem
  Electrical Reference : fl_lib/Electrical/Electrical Elements/Electrical Reference
  PS Three-Element Demux : fl_lib/Physical Signals/Nonlinear Operators/PS Three-Element Demux
      settings: InternalSimscapePortConfiguration="{\"Bottom\":[],\"Left\":[{\"id\":\"abc\",\"label\":\"abc\",\"type\":\"input\"}],\"Right\":[{\"id\":\"a\",\"label\":\"a\",\"type\":\"output\"},{\"id\":\"b\",\"label\":\"b\",\"type\":\"output\"},{\"id\":\"c\",\"label\":\"c\",\"type\":\"output\"}],\"Top\":[]}"
      settings: LibrarySourceBlock=|
      | ee_lib/Connectors &
      | References/PS Three-Element Demux
  PS-Simulink Converter : nesl_utility/PS-Simulink Converter  PhysicalDomain=network_engine_domain  SubClassName=ps_output  LeftPortType=input  RightPortType=output  PseudoPeriodic=off  Frequencies=[]  VectorFormat=inherit  Unit=inherit  AffineConversion=off
  Phase Splitter : ee_lib/Connectors & References/Phase Splitter
  Simulink-PS Converter : nesl_utility/Simulink-PS Converter  PhysicalDomain=network_engine_domain  SubClassName=ps_input  LeftPortType=input  RightPortType=output  PseudoPeriodic=off  Frequencies=[]  NoiseDistribution=none  NoiseParameters=[]  Unit=1  AffineConversion=off  FilteringAndDerivatives=provide  SimscapeFilterOrder=1  InputFilterTimeConstant=0.001  UdotUserProvided=0
  Simulink-PS Converter1 : nesl_utility/Simulink-PS Converter  PhysicalDomain=network_engine_domain  SubClassName=ps_input  LeftPortType=input  RightPortType=output  PseudoPeriodic=off  Frequencies=[]  NoiseDistribution=none  NoiseParameters=[]  Unit=1  AffineConversion=off  FilteringAndDerivatives=provide  SimscapeFilterOrder=1  InputFilterTimeConstant=0.001  UdotUserProvided=0
  Switch : fl_lib/Electrical/Electrical Elements/Switch  R_closed=0.01 Ohm  G_open=1e-8 1/Ohm  Threshold=0.5  i_specify=off  i_priority=None  i=0 A  i_nominal_specify=off  i_nominal_unit=A  i_nominal_value=1  v_specify=off  v_priority=None  v=0 V  v_nominal_specify=off  v_nominal_unit=V  v_nominal_value=1
  Switch1 : fl_lib/Electrical/Electrical Elements/Switch  R_closed=0.01 Ohm  G_open=1e-8 1/Ohm  Threshold=0.5  i_specify=off  i_priority=None  i=0 A  i_nominal_specify=off  i_nominal_unit=A  i_nominal_value=1  v_specify=off  v_priority=None  v=0 V  v_nominal_specify=off  v_nominal_unit=V  v_nominal_value=1
  Switch2 : fl_lib/Electrical/Electrical Elements/Switch  R_closed=0.01 Ohm  G_open=1e-8 1/Ohm  Threshold=0.5  i_specify=off  i_priority=None  i=0 A  i_nominal_specify=off  i_nominal_unit=A  i_nominal_value=1  v_specify=off  v_priority=None  v=0 V  v_nominal_specify=off  v_nominal_unit=V  v_nominal_value=1
  Vabc : PMIOPort  Side=Right
  Iabc : Outport
  wires:
  PS-Simulink Converter/1 -> Iabc/1
  Gates_DutyCycle/1 -> DutyCycles2Levels/1(DutyCycles)
  DutyCycles2Levels/1(Dabc) -> Average-Value Inverter/1
  DutyCycles2Levels/2(BridgeHighImpedance) -> Simulink-PS Converter1/1
  Average-Value Inverter/1 -> Simulink-PS Converter/1
  Constant/1 -> Average-Value Inverter/2
  connections:
  Vabc/RConn1 -- Current Sensor (Three-Phase)/RConn2
  PS-Simulink Converter/LConn1 -- Current Sensor (Three-Phase)/RConn1
  DC Voltage Source/RConn1 -- Controlled Voltage Source (Three-Phase)/LConn2 -- Electrical Reference/LConn1 -- Diode4/LConn1 -- Diode5/LConn1 -- Diode3/LConn1
  Switch/RConn2 -- Controlled Voltage Source (Three-Phase)/RConn1
  Switch1/RConn2 -- Controlled Voltage Source (Three-Phase)/RConn2
  Switch2/RConn2 -- Controlled Voltage Source (Three-Phase)/RConn3
  DC Voltage Source/LConn1 -- Diode1/RConn1 -- Diode2/RConn1 -- Diode/RConn1
  Phase Splitter/LConn1 -- Current Sensor (Three-Phase)/LConn1
  Diode/LConn1 -- Phase Splitter/RConn1 -- Switch/LConn1 -- Diode3/RConn1
  Diode1/LConn1 -- Phase Splitter/RConn2 -- Switch1/LConn1 -- Diode4/RConn1
  Diode2/LConn1 -- Phase Splitter/RConn3 -- Switch2/LConn1 -- Diode5/RConn1
  PS Three-Element Demux/LConn1 -- Simulink-PS Converter1/RConn1
  PS Three-Element Demux/RConn1 -- Switch/RConn1
  Switch1/RConn1 -- PS Three-Element Demux/RConn2
  Switch2/RConn1 -- PS Three-Element Demux/RConn3
  Simulink-PS Converter/RConn1 -- Controlled Voltage Source (Three-Phase)/LConn1

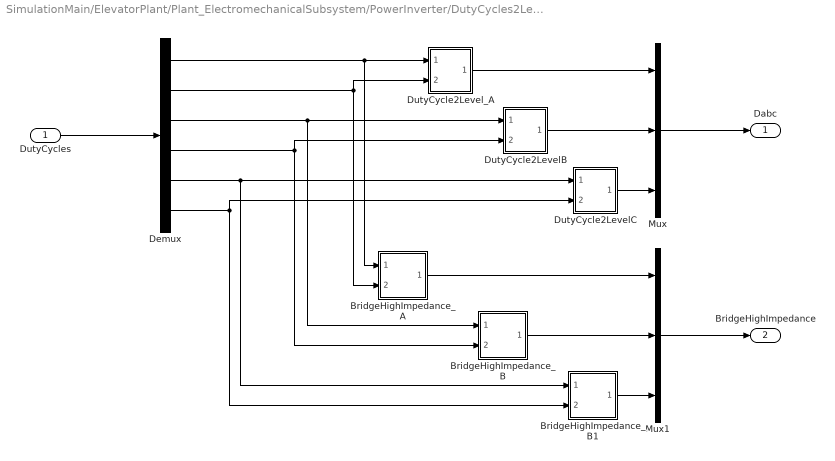
== system SimulationMain/ElevatorPlant/Plant_ElectromechanicalSubsystem/PowerInverter/DutyCycles2Levels ==
  DutyCycles : Inport
  BridgeHighImpedance_A : Subsystem  ReferencedSubsystem=DutyCycle2BridgeImpedance
  BridgeHighImpedance_B : Subsystem  ReferencedSubsystem=DutyCycle2BridgeImpedance
  BridgeHighImpedance_B1 : Subsystem  ReferencedSubsystem=DutyCycle2BridgeImpedance
  Demux : Demux  Outputs=6
  DutyCycle2LevelB : Subsystem  TreatAsAtomicUnit=on  ReferencedSubsystem=DutyCycle2_Level
  DutyCycle2LevelC : Subsystem  TreatAsAtomicUnit=on  ReferencedSubsystem=DutyCycle2_Level
  DutyCycle2Level_A : Subsystem  TreatAsAtomicUnit=on  ReferencedSubsystem=DutyCycle2_Level
  Mux : Mux  Inputs=3
  Mux1 : Mux  Inputs=3
  Dabc : Outport
  BridgeHighImpedance : Outport  Port=2
  wires:
  DutyCycles/1 -> Demux/1
  Demux/1 -> DutyCycle2Level_A/1, BridgeHighImpedance_A/1
  Demux/2 -> DutyCycle2Level_A/2, BridgeHighImpedance_A/2
  Demux/3 -> BridgeHighImpedance_B/1, DutyCycle2LevelB/1
  Demux/4 -> DutyCycle2LevelB/2, BridgeHighImpedance_B/2
  Demux/6 -> DutyCycle2LevelC/2, BridgeHighImpedance_B1/2
  Demux/5 -> BridgeHighImpedance_B1/1, DutyCycle2LevelC/1
  DutyCycle2LevelC/1 -> Mux/3
  DutyCycle2LevelB/1 -> Mux/2
  DutyCycle2Level_A/1 -> Mux/1
  BridgeHighImpedance_A/1 -> Mux1/1
  BridgeHighImpedance_B/1 -> Mux1/2
  BridgeHighImpedance_B1/1 -> Mux1/3
  Mux1/1 -> BridgeHighImpedance/1
  Mux/1 -> Dabc/1

== matlab function SimulationMain/Elevator Floor Input/MATLAB Function ==
  data: t input; v_t output; total_dis input; a input; v_const input; StepTime input
function v_t= fcn(t,total_dis,a,v_const,StepTime)
% Equation for Elevator Velocity :
% v(t) = v0 + (vf-v0)*((t-t0)/(tf-t0))^2;
% Max Elevator acceleration a = 1 m/s^2; 
% Height of One Floor = 3.60m 
% Rated Max Constant Velocity of the Elevator = 1.5m/s
% Total Distance Travelled = v^2/2a + v*(t2-t1) + v^2/2a ; 

% t1 = v/a; % Period of Non-zero Acceleration
% t1 to t2 ; Period of Constant Velocity
% t2 = (TotalDistance - v^2/a)/v + t1;
% tf-t2 = t1; % Period of Non-zero De-Acceleration

if t>StepTime
    t = t-StepTime;
end

if t <= (v_const/a)
    v0 = 0;
    t0 = 0;
    tf = (v_const/a);
    vf = v_const;
     
elseif t > (v_const/a) && t <= (total_dis - (v_const^2)/a)/v_const + (v_const/a)
       vf = v_const;
       v0 = v_const;
       t0 = (v_const/a);
       tf = (total_dis - (v_const^2)/a)/v_const + (v_const/a);
       
elseif  t > (total_dis - (v_const^2)/a)/v_const + (v_const/a) &&...
        t <= ((v_const/a) + (total_dis - (v_const^2)/a)/v_const + (v_const/a))
    
    tf = (v_const/a) + (total_dis - (v_const^2)/a)/v_const + (v_const/a);
    t0 = (total_dis - (v_const^2)/a)/v_const + (v_const/a);
    vf = 0 ;
    v0 = v_const;   
else
   
    vf = 0;
    v0 = 0;
    t0 = 0;
    tf = (v_const/a) + (total_dis - (v_const^2)/a)/v_const + (v_const/a);
end

v_t = v0 + (vf-v0)*(((t-t0)/(tf-t0))^2)*(3 - 2*((t-t0)/(tf-t0)));

end
